simulink model "hrg_wa_v4_bitstream"  (R2025a)
settings: Solver=ode4  StartTime=0.0  StopTime=wl_stop  FixedStep=wl_Tp  RelTol=1e-3
PostLoadFcn:
  | addpath(fileparts(fileparts(get_param('hrg_wa_v4_bitstream','FileName')))); wl_setup(getVariable(get_param('hrg_wa_v4_bitstream','ModelWorkspace'),'wl_saved_configuration'));
model workspace (MAT data in the model file):
  wl_saved_configuration.stage = 4
  wl_saved_configuration.name = 'hrg_wa_v4_bitstream'
  wl_saved_configuration.head.sourceProfile = 'C:\Users\11725\Desktop\HRG_WA\HRG_WA_simulink\..\HRG_WA_Digital_ASIC_MATLAB_v4_6_5_FRP_validation_fix\HRG_WA\config\head_default.json'
  wl_saved_configuration.head.measurementStatus = 'assumed, not a measured head'
  wl_saved_configuration.head.f0 = 5000
  wl_saved_configuration.head.Q = 2000000
  wl_saved_configuration.head.bryan = 0.277
  wl_saved_configuration.head.gamma = 0.00785398163397
  wl_saved_configuration.head.dgamma = 0.00025
  wl_saved_configuration.head.dampingAxis = 0.296705972839
  wl_saved_configuration.head.splitHz = 0.008
  wl_saved_configuration.head.stiffnessAxis = 0.715584993318
  wl_saved_configuration.head.detuningHz = 0
  wl_saved_configuration.head.duffingHz = 0.015
  wl_saved_configuration.head.temperatureCoeff = -1.8e-05
  wl_saved_configuration.head.referenceTemperature = 25
  wl_saved_configuration.head.detect = [1  0.003; -0.002  1]
  wl_saved_configuration.head.detectPhase = [0; 0]
  wl_saved_configuration.head.drive = [1  0; 0  1]
  wl_saved_configuration.head.detectCubic = 0
  wl_saved_configuration.head.iqBits = 0
  wl_saved_configuration.head.iqFullScale = 2
  wl_saved_configuration.head.energyTarget = 1
  wl_saved_configuration.head.initialEnergy = 1
  wl_saved_configuration.head.initialTheta = 0.13962634016
  wl_saved_configuration.head.initialQuadRatio = 0
  wl_saved_configuration.head.energyKp = 0.8
  wl_saved_configuration.head.energyKi = 0.4
  wl_saved_configuration.head.quadKp = 2
  wl_saved_configuration.head.quadKi = 1
  wl_saved_configuration.head.pllKp = 0.8
  wl_saved_configuration.head.pllKi = 1
  wl_saved_configuration.head.energyLimit = 1
  wl_saved_configuration.head.quadLimit = 1
  wl_saved_configuration.head.pllLimitHz = 2
  wl_saved_configuration.head.antiWindup = 5
  wl_saved_configuration.head.loopEnable = 1
  wl_saved_configuration.head.Ts = 0.001
  wl_saved_configuration.head.rateTau = 0.00353677651315
  wl_saved_configuration.head.energyThreshold = 0.02
  wl_saved_configuration.head.angleThreshold = 0.01
  wl_saved_configuration.head.duration = 12
  wl_saved_configuration.head.omega = 1.3962634016
  wl_saved_configuration.head.virtualRate = 0
  wl_saved_configuration.head.temperature = 25
  wl_saved_configuration.head.fullStep = 2e-06
  wl_saved_configuration.fsAdc = 160000
  wl_saved_configuration.fsPlant = 640000
  wl_saved_configuration.duration = 0.04
  wl_saved_configuration.seed = 20261021
  wl_saved_configuration.massKg = 1e-06
  wl_saved_configuration.displacementM = 1e-07
  wl_saved_configuration.gapM = 5e-06
  wl_saved_configuration.c0F = 1e-12
  wl_saved_configuration.cfF = 1e-12
  wl_saved_configuration.rfOhm = 1000000000
  wl_saved_configuration.biasV = 10
  wl_saved_configuration.cvBandwidthHz = 30000
  wl_saved_configuration.pgaBandwidthHz = 30000
  wl_saved_configuration.pgaGain = 1
  wl_saved_configuration.cvEnVrtHz = 1e-08
  wl_saved_configuration.cvInArtHz = 1e-14
  wl_saved_configuration.temperatureK = 298.15
  wl_saved_configuration.pgaNoiseVrtHz = 1e-08
  wl_saved_configuration.afeOffsetV = [0; 0]
  wl_saved_configuration.afeLimitV = 1.8
  wl_saved_configuration.adcBits = 18
  wl_saved_configuration.adcFsV = 2
  wl_saved_configuration.adcOffsetV = [0; 0]
  wl_saved_configuration.adcGain = [1; 1]
  wl_saved_configuration.adcInlCubic = 0
  wl_saved_configuration.jitterRmsS = 2e-09
  wl_saved_configuration.channelSkewS = 0
  wl_saved_configuration.adcDelay = 1
  wl_saved_configuration.adcArchitecture = 'sigma_delta'
  wl_saved_configuration.cicStages = 3
  wl_saved_configuration.fir = [0.111111111111 0.222222222222 0.333333333333 0.222222222222 0.111111111111]
  wl_saved_configuration.dacBits = 16
  wl_saved_configuration.dacFsV = 2
  wl_saved_configuration.dacDelay = 1
  wl_saved_configuration.dacInlCubic = 0
  wl_saved_configuration.dacArchitecture = 'sigma_delta'
  wl_saved_configuration.driveNPerV = 1e-07
  wl_saved_configuration.driverBandwidthHz = 50000
  wl_saved_configuration.driverGain = [1; 1]
  wl_saved_configuration.driverSlewVPerS = 200000
  wl_saved_configuration.driverNoiseVrtHz = 2e-08
  wl_saved_configuration.driverLimitV = 1.8
  wl_saved_configuration.feedthroughF = 0
  wl_saved_configuration.pipelineCtrl = 3
  wl_saved_configuration.iqFractionBits = 22
  wl_saved_configuration.controlFractionBits = 22
  wl_saved_configuration.antiAliasHz = 18000
  wl_saved_configuration.noiseEnable = 1
  wl_saved_configuration.circuitEnable = 1
  wl_saved_configuration.kalman = 0
  wl_saved_configuration.online = 0
  wl_saved_configuration.frp = 0
  wl_saved_configuration.calibrationPermit = 0
  wl_saved_configuration.frpSequence = 0
  wl_saved_configuration.frpFreeze = 0
  wl_saved_configuration.frpTheta = [0; 0; 0; 0; 0; 0; 0; 0; 0]
  wl_saved_configuration.matrixApply = 0
  wl_saved_configuration.compensationApply = 0
  wl_saved_configuration.temperatureCompensate = 0
  wl_saved_configuration.temperatureBiasCoefficients = [0; 0; 0]
  wl_saved_configuration.zeroRateCertified = 0
  wl_saved_configuration.virtualRate = 0
  wl_saved_configuration.inputRate = 1.3962634016
  wl_saved_configuration.inputFrequencyHz = 0
  wl_saved_configuration.inputRateAmplitude = 0
  wl_saved_configuration.temperatureC = 25
  wl_saved_configuration.temperatureRampCPerS = 0
  wl_saved_configuration.observers = 0
  wl_saved_configuration.spectra = 0
  wl_saved_configuration.maxLogPoints = 80000
  wl_saved_configuration.sdmLeak = 0.9999
  wl_saved_configuration.sdmReferenceV = 2
  wl_saved_configuration.tdmEnable = 0
  wl_saved_configuration.knownPhaseCalibrationRad = -2.63258802151
  wl_saved_configuration.virtualGainCalibration = 1.10062721786
  wl_saved_configuration.learnStartS = 0.25
  wl_saved_configuration.measurementStatus = 'assumed'
  wl_saved_configuration.scope = 'Behavioral circuit interfaces, not transistor or bit-true RTL signoff'
  wl_saved_configuration.cvEquivalentNoiseVrtHz = 3.43925722091e-07
undefined symbols (not defined in the file): wl_boxcar, wl_brownVariance, wl_c, wl_capacitance, wl_control_tick, wl_cvGain, wl_cvNoiseVariance, wl_cvTau, wl_D, wl_detectGain, wl_driverNoiseVariance, wl_fir, wl_forceGain, wl_hToV, wl_input, wl_iq_quantize, wl_J, wl_jitterVariance, wl_K, wl_mix, wl_modulate, wl_p, wl_pgaNoiseVariance, wl_q0, wl_R, wl_Ta, wl_Tc, wl_Tp, wl_v0
settings Model: Creator=11725  LastModifiedBy=11725
settings DataIOCC: SaveOutput=off
settings DebuggingCC: SignalInfNanChecking=error  AlgebraicLoopMsg=error

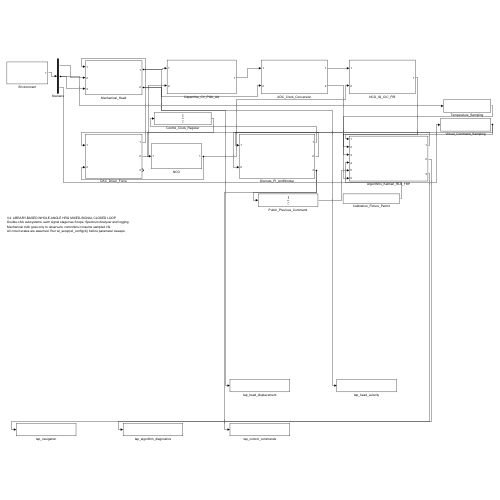
[thumbnail: Simulink's stored preview of the top-level diagram]
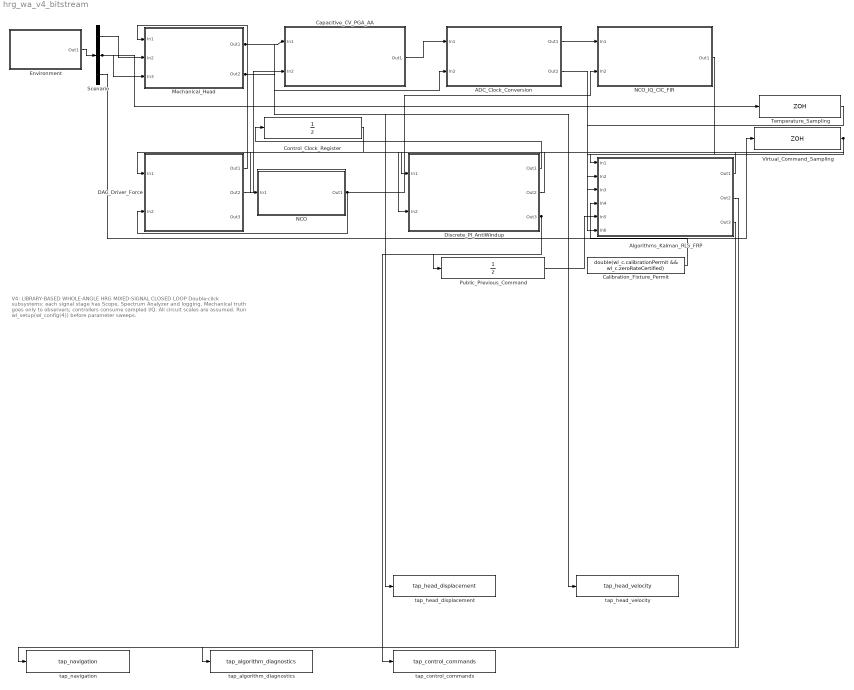
== system hrg_wa_v4_bitstream ==
  note: V4: LIBRARY-BASED WHOLE-ANGLE HRG MIXED-SIGNAL CLOSED LOOP
      | Double-click subsystems: each signal stage has Scope, Spectrum Analyzer and logging.
      | Mechanical truth goes only to observers; controllers consume sampled I/Q.
      | All circuit scales are assumed. Run wl_setup(wl_config(4)) before parameter sweeps.
  ADC_Clock_Conversion : Subsystem
  Algorithms_Kalman_RLS_FRP : Subsystem
  Calibration_Fixture_Permit : Constant  Value=double(wl_c.calibrationPermit && wl_c.zeroRateCertified)
  Capacitive_CV_PGA_AA : Subsystem
  Control_Clock_Register : UnitDelay  InitialCondition=zeros(4,1)  SampleTime=wl_Tc  HasFrameUpgradeWarning=on
  DAC_Driver_Force : Subsystem
  Discrete_PI_AntiWindup : Subsystem
  Environment : Subsystem
  Mechanical_Head : Subsystem
  NCO : Subsystem
  NCO_IQ_CIC_FIR : Subsystem
  Public_Previous_Command : UnitDelay  InitialCondition=zeros(3,1)  SampleTime=wl_Tc  HasFrameUpgradeWarning=on
  Scenario : Demux  Outputs=[2 1 1]
  Temperature_Sampling : ZeroOrderHold  SampleTime=wl_Tc
  Virtual_Command_Sampling : ZeroOrderHold  SampleTime=wl_Tc
  tap_algorithm_diagnostics : ToWorkspace  VariableName=tap_algorithm_diagnostics  SaveFormat=Timeseries  SampleTime=-1
      settings: MaxDataPoints=80000
  tap_control_commands : ToWorkspace  VariableName=tap_control_commands  SaveFormat=Timeseries  SampleTime=-1
      settings: MaxDataPoints=80000
  tap_head_displacement : ToWorkspace  VariableName=tap_head_displacement  SaveFormat=Timeseries  SampleTime=-1
      settings: MaxDataPoints=80000
  tap_head_velocity : ToWorkspace  VariableName=tap_head_velocity  SaveFormat=Timeseries  SampleTime=-1
      settings: MaxDataPoints=80000
  tap_navigation : ToWorkspace  VariableName=tap_navigation  SaveFormat=Timeseries  SampleTime=-1
      settings: MaxDataPoints=80000
  wires:
  Environment/1(Out1) -> Scenario/1
  Scenario/1 -> Mechanical_Head/2(In2)
  Scenario/2 -> Mechanical_Head/3(In3), Temperature_Sampling/1
  DAC_Driver_Force/1(Out1) -> Mechanical_Head/1(In1)
  Mechanical_Head/1(Out1) -> Capacitive_CV_PGA_AA/1(In1), tap_head_displacement/1
  DAC_Driver_Force/2(Out2) -> Capacitive_CV_PGA_AA/2(In2)
  Capacitive_CV_PGA_AA/1(Out1) -> ADC_Clock_Conversion/1(In1)
  Mechanical_Head/2(Out2) -> ADC_Clock_Conversion/2(In2), tap_head_velocity/1
  ADC_Clock_Conversion/1(Out1) -> NCO_IQ_CIC_FIR/1(In1)
  NCO/1(Out1) -> NCO_IQ_CIC_FIR/2(In2), DAC_Driver_Force/2(In2)
  NCO_IQ_CIC_FIR/1(Out1) -> Algorithms_Kalman_RLS_FRP/1(In1)
  Scenario/3 -> Virtual_Command_Sampling/1
  Temperature_Sampling/1 -> Algorithms_Kalman_RLS_FRP/2(In2)
  Virtual_Command_Sampling/1 -> Algorithms_Kalman_RLS_FRP/3(In3), Discrete_PI_AntiWindup/2(In2)
  Calibration_Fixture_Permit/1 -> Algorithms_Kalman_RLS_FRP/4(In4)
  Discrete_PI_AntiWindup/3(Out3) -> Public_Previous_Command/1, tap_control_commands/1
  Public_Previous_Command/1 -> Algorithms_Kalman_RLS_FRP/5(In5)
  Algorithms_Kalman_RLS_FRP/1(Out1) -> Discrete_PI_AntiWindup/1(In1)
  Discrete_PI_AntiWindup/2(Out2) -> NCO/1(In1)
  Discrete_PI_AntiWindup/1(Out1) -> Control_Clock_Register/1
  Control_Clock_Register/1 -> DAC_Driver_Force/1(In1)
  ADC_Clock_Conversion/2(Out2) -> Algorithms_Kalman_RLS_FRP/6(In6)
  Algorithms_Kalman_RLS_FRP/2(Out2) -> tap_navigation/1
  Algorithms_Kalman_RLS_FRP/3(Out3) -> tap_algorithm_diagnostics/1

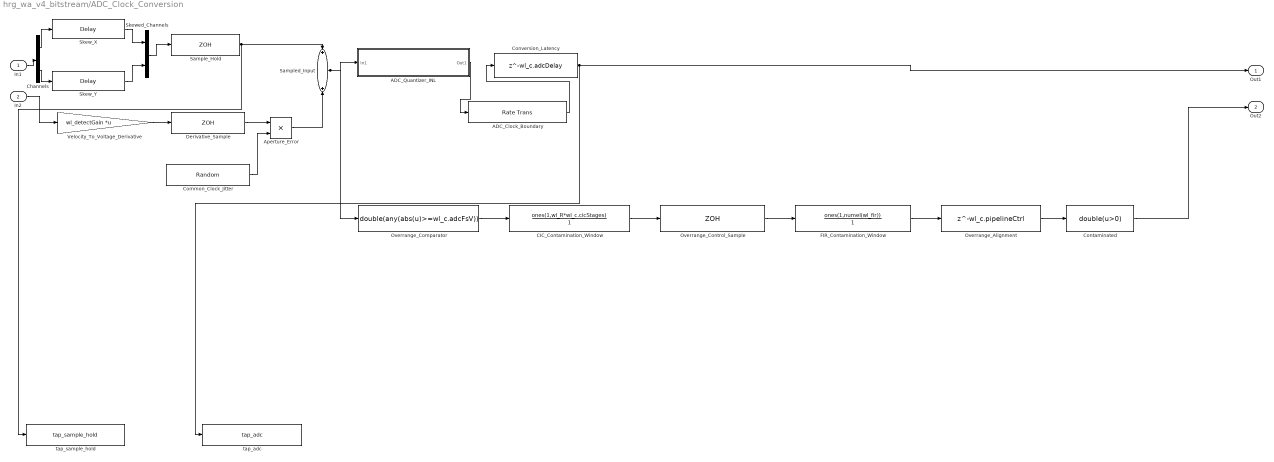
== system hrg_wa_v4_bitstream/ADC_Clock_Conversion ==
  In1 : Inport
  In2 : Inport  Port=2
  ADC_Clock_Boundary : RateTransition  Integrity=off  Deterministic=off  OutPortSampleTime=wl_Ta
  ADC_Quantizer_INL : Subsystem
  Aperture_Error : Product
  CIC_Contamination_Window : DiscreteFilter  Numerator=ones(1,wl_R*wl_c.cicStages)  Denominator=1  SampleTime=wl_Ta
  Channels : Demux  Outputs=2
  Common_Clock_Jitter : RandomNumber  Variance=wl_jitterVariance  Seed=wl_c.seed+621  SampleTime=wl_Ta
  Contaminated : MATLABFcn  MATLABFcn=double(u>0)  OutputDimensions=1
  Conversion_Latency : Delay  DelayLength=wl_c.adcDelay  InitialCondition=0  SampleTime=wl_Ta
  Derivative_Sample : ZeroOrderHold  SampleTime=wl_Ta
  FIR_Contamination_Window : DiscreteFilter  Numerator=ones(1,numel(wl_fir))  Denominator=1  SampleTime=wl_Tc
  Overrange_Alignment : Delay  DelayLength=wl_c.pipelineCtrl  InitialCondition=0  SampleTime=wl_Tc
  Overrange_Comparator : MATLABFcn  MATLABFcn=double(any(abs(u)>=wl_c.adcFsV))  OutputDimensions=1
  Overrange_Control_Sample : ZeroOrderHold  SampleTime=wl_Tc
  Sample_Hold : ZeroOrderHold  SampleTime=wl_Ta
  Sampled_Input : Sum
  Skew_X : TransportDelay  DelayTime=max(-wl_c.channelSkewS,0)
  Skew_Y : TransportDelay  DelayTime=max(wl_c.channelSkewS,0)
  Skewed_Channels : Mux  Inputs=2
  Velocity_To_Voltage_Derivative : Gain  Gain=wl_detectGain  Multiplication=Matrix(K*u)
  tap_adc : ToWorkspace  VariableName=tap_adc  SaveFormat=Timeseries  SampleTime=-1
      settings: MaxDataPoints=80000
  tap_sample_hold : ToWorkspace  VariableName=tap_sample_hold  SaveFormat=Timeseries  SampleTime=-1
      settings: MaxDataPoints=80000
  Out1 : Outport
  Out2 : Outport  Port=2
  wires:
  In1/1 -> Channels/1
  Channels/1 -> Skew_X/1
  Channels/2 -> Skew_Y/1
  Skew_X/1 -> Skewed_Channels/1
  Skew_Y/1 -> Skewed_Channels/2
  Skewed_Channels/1 -> Sample_Hold/1
  In2/1 -> Velocity_To_Voltage_Derivative/1
  Velocity_To_Voltage_Derivative/1 -> Derivative_Sample/1
  Derivative_Sample/1 -> Aperture_Error/1
  Common_Clock_Jitter/1 -> Aperture_Error/2
  Sample_Hold/1 -> Sampled_Input/1, tap_sample_hold/1
  Aperture_Error/1 -> Sampled_Input/2
  Sampled_Input/1 -> ADC_Quantizer_INL/1(In1), Overrange_Comparator/1
  ADC_Quantizer_INL/1(Out1) -> ADC_Clock_Boundary/1
  ADC_Clock_Boundary/1 -> Conversion_Latency/1
  Conversion_Latency/1 -> Out1/1, tap_adc/1
  Overrange_Comparator/1 -> CIC_Contamination_Window/1
  CIC_Contamination_Window/1 -> Overrange_Control_Sample/1
  Overrange_Control_Sample/1 -> FIR_Contamination_Window/1
  FIR_Contamination_Window/1 -> Overrange_Alignment/1
  Overrange_Alignment/1 -> Contaminated/1
  Contaminated/1 -> Out2/1

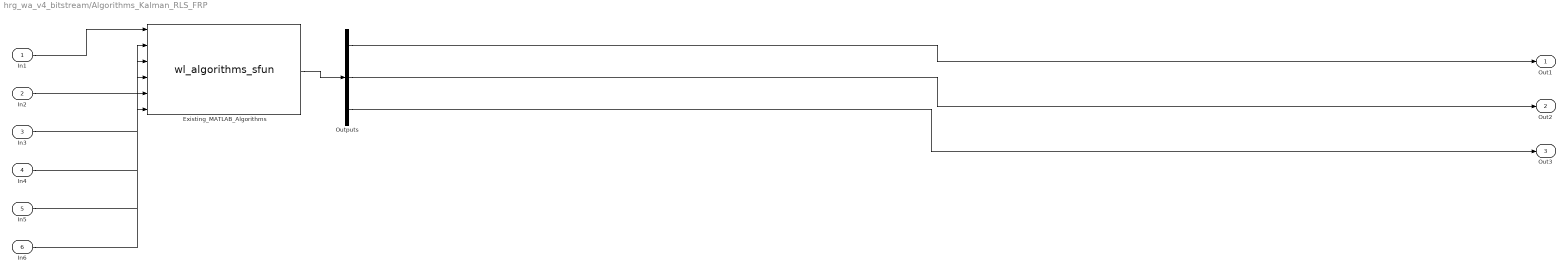
== system hrg_wa_v4_bitstream/Algorithms_Kalman_RLS_FRP ==
  In1 : Inport
  In2 : Inport  Port=2
  In3 : Inport  Port=3
  In4 : Inport  Port=4
  In5 : Inport  Port=5
  In6 : Inport  Port=6
  Existing_MATLAB_Algorithms : M-S-Function  FunctionName=wl_algorithms_sfun  Parameters=wl_c
  Outputs : Demux  Outputs=[10 4 21]
  Out1 : Outport
  Out2 : Outport  Port=2
  Out3 : Outport  Port=3
  wires:
  In1/1 -> Existing_MATLAB_Algorithms/1
  In2/1 -> Existing_MATLAB_Algorithms/2
  In3/1 -> Existing_MATLAB_Algorithms/3
  In4/1 -> Existing_MATLAB_Algorithms/4
  In5/1 -> Existing_MATLAB_Algorithms/5
  In6/1 -> Existing_MATLAB_Algorithms/6
  Existing_MATLAB_Algorithms/1 -> Outputs/1
  Outputs/1 -> Out1/1
  Outputs/2 -> Out2/1
  Outputs/3 -> Out3/1

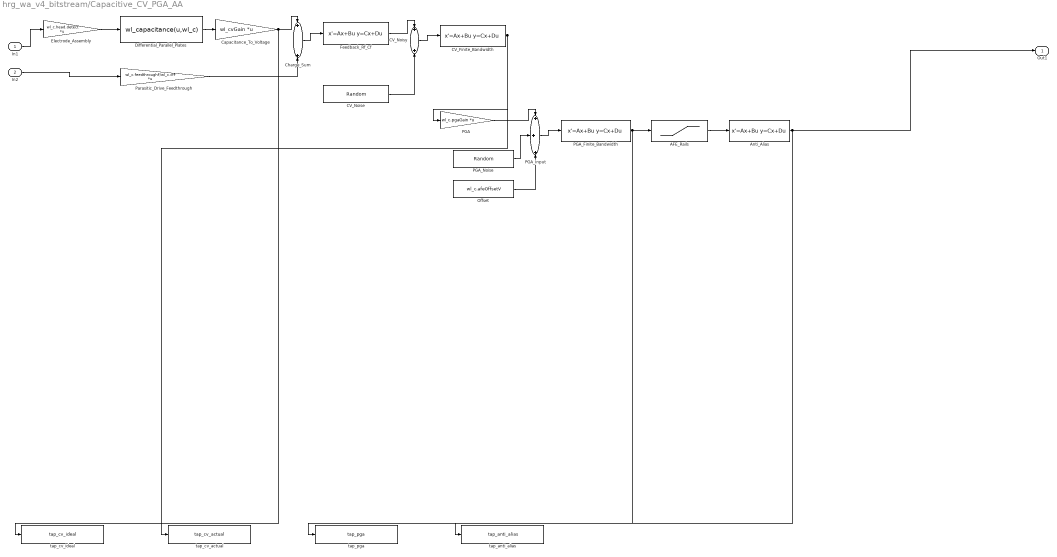
== system hrg_wa_v4_bitstream/Capacitive_CV_PGA_AA ==
  In1 : Inport
  In2 : Inport  Port=2
  AFE_Rails : Saturate  UpperLimit=wl_c.afeLimitV  LowerLimit=-wl_c.afeLimitV
  Anti_Alias : StateSpace  A=-2*pi*wl_c.antiAliasHz*eye(2)  B=2*pi*wl_c.antiAliasHz*eye(2)  C=eye(2)  D=zeros(2)  InitialCondition=0
  CV_Finite_Bandwidth : StateSpace  A=-2*pi*wl_c.cvBandwidthHz*eye(2)  B=2*pi*wl_c.cvBandwidthHz*eye(2)  C=eye(2)  D=zeros(2)  InitialCondition=0
  CV_Noise : RandomNumber  Mean=[0;0]  Variance=wl_cvNoiseVariance*[1;1]  Seed=[wl_c.seed+601;wl_c.seed+602]  SampleTime=wl_Tp
  CV_Noisy : Sum
  Capacitance_To_Voltage : Gain  Gain=wl_cvGain  Multiplication=Matrix(K*u)
  Charge_Sum : Sum
  Differential_Parallel_Plates : MATLABFcn  MATLABFcn=wl_capacitance(u,wl_c)  OutputDimensions=2
  Electrode_Assembly : Gain  Gain=wl_c.head.detect  Multiplication=Matrix(K*u)
  Feedback_Rf_Cf : StateSpace  A=-eye(2)/wl_cvTau  B=eye(2)/wl_cvTau  C=-eye(2)  D=eye(2)  InitialCondition=0
  Offset : Constant  Value=wl_c.afeOffsetV
  PGA : Gain  Gain=wl_c.pgaGain  Multiplication=Matrix(K*u)
  PGA_Finite_Bandwidth : StateSpace  A=-2*pi*wl_c.pgaBandwidthHz*eye(2)  B=2*pi*wl_c.pgaBandwidthHz*eye(2)  C=eye(2)  D=zeros(2)  InitialCondition=0
  PGA_Input : Sum  Inputs=+++
  PGA_Noise : RandomNumber  Mean=[0;0]  Variance=wl_pgaNoiseVariance*[1;1]  Seed=[wl_c.seed+611;wl_c.seed+612]  SampleTime=wl_Tp
  Parasitic_Drive_Feedthrough : Gain  Gain=wl_c.feedthroughF/wl_c.cfF  Multiplication=Matrix(K*u)
  tap_anti_alias : ToWorkspace  VariableName=tap_anti_alias  SaveFormat=Timeseries  SampleTime=-1
      settings: MaxDataPoints=80000
  tap_cv_actual : ToWorkspace  VariableName=tap_cv_actual  SaveFormat=Timeseries  SampleTime=-1
      settings: MaxDataPoints=80000
  tap_cv_ideal : ToWorkspace  VariableName=tap_cv_ideal  SaveFormat=Timeseries  SampleTime=-1
      settings: MaxDataPoints=80000
  tap_pga : ToWorkspace  VariableName=tap_pga  SaveFormat=Timeseries  SampleTime=-1
      settings: MaxDataPoints=80000
  Out1 : Outport
  wires:
  In1/1 -> Electrode_Assembly/1
  Electrode_Assembly/1 -> Differential_Parallel_Plates/1
  Differential_Parallel_Plates/1 -> Capacitance_To_Voltage/1
  In2/1 -> Parasitic_Drive_Feedthrough/1
  Capacitance_To_Voltage/1 -> Charge_Sum/1, tap_cv_ideal/1
  Parasitic_Drive_Feedthrough/1 -> Charge_Sum/2
  Charge_Sum/1 -> Feedback_Rf_Cf/1
  Feedback_Rf_Cf/1 -> CV_Noisy/1
  CV_Noise/1 -> CV_Noisy/2
  CV_Noisy/1 -> CV_Finite_Bandwidth/1
  CV_Finite_Bandwidth/1 -> PGA/1, tap_cv_actual/1
  PGA/1 -> PGA_Input/1
  PGA_Noise/1 -> PGA_Input/2
  Offset/1 -> PGA_Input/3
  PGA_Input/1 -> PGA_Finite_Bandwidth/1
  PGA_Finite_Bandwidth/1 -> AFE_Rails/1, tap_pga/1
  AFE_Rails/1 -> Anti_Alias/1
  Anti_Alias/1 -> Out1/1, tap_anti_alias/1

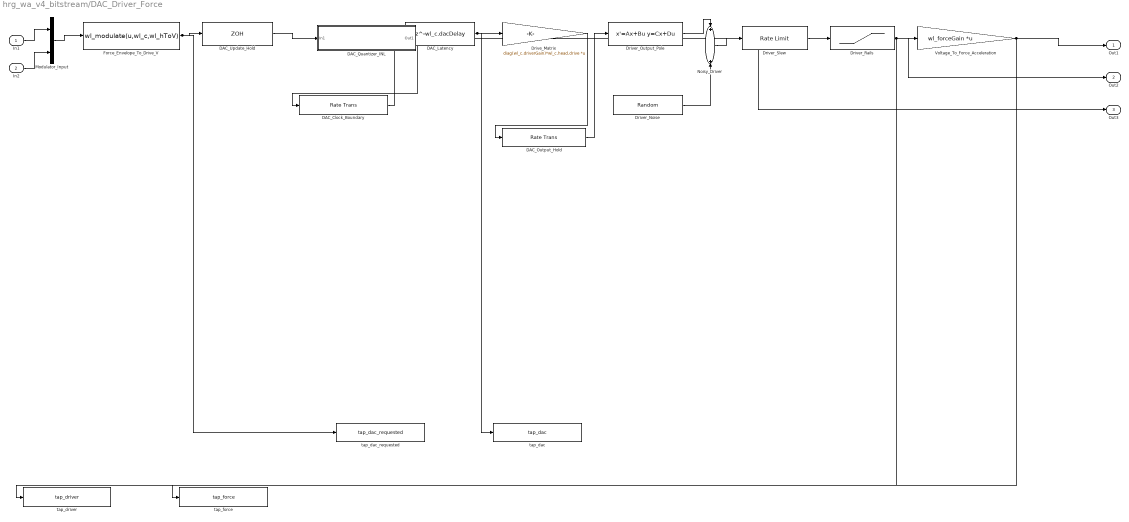
== system hrg_wa_v4_bitstream/DAC_Driver_Force ==
  In1 : Inport
  In2 : Inport  Port=2
  DAC_Clock_Boundary : RateTransition  Integrity=off  Deterministic=off  OutPortSampleTime=wl_Ta
  DAC_Latency : Delay  DelayLength=wl_c.dacDelay  InitialCondition=0  SampleTime=wl_Ta
  DAC_Output_Hold : RateTransition  Integrity=off  Deterministic=off  OutPortSampleTime=0
  DAC_Quantizer_INL : Subsystem
  DAC_Update_Hold : ZeroOrderHold  SampleTime=wl_Ta
  Drive_Matrix : Gain  Gain=diag(wl_c.driverGain)*wl_c.head.drive  Multiplication=Matrix(K*u)
  Driver_Noise : RandomNumber  Mean=[0;0]  Variance=wl_driverNoiseVariance*[1;1]  Seed=[wl_c.seed+631;wl_c.seed+632]  SampleTime=wl_Tp
  Driver_Output_Pole : StateSpace  A=-2*pi*wl_c.driverBandwidthHz*eye(2)  B=2*pi*wl_c.driverBandwidthHz*eye(2)  C=eye(2)  D=zeros(2)  InitialCondition=0
  Driver_Rails : Saturate  UpperLimit=wl_c.driverLimitV  LowerLimit=-wl_c.driverLimitV
  Driver_Slew : RateLimiter  RisingSlewLimit=wl_c.driverSlewVPerS  FallingSlewLimit=-wl_c.driverSlewVPerS  SampleTimeMode=inherited
  Force_Envelope_To_Drive_V : MATLABFcn  MATLABFcn=wl_modulate(u,wl_c,wl_hToV)  OutputDimensions=2
  Modulator_Input : Mux  Inputs=2
  Noisy_Driver : Sum
  Voltage_To_Force_Acceleration : Gain  Gain=wl_forceGain  Multiplication=Matrix(K*u)
  tap_dac : ToWorkspace  VariableName=tap_dac  SaveFormat=Timeseries  SampleTime=-1
      settings: MaxDataPoints=80000
  tap_dac_requested : ToWorkspace  VariableName=tap_dac_requested  SaveFormat=Timeseries  SampleTime=-1
      settings: MaxDataPoints=80000
  tap_driver : ToWorkspace  VariableName=tap_driver  SaveFormat=Timeseries  SampleTime=-1
      settings: MaxDataPoints=80000
  tap_force : ToWorkspace  VariableName=tap_force  SaveFormat=Timeseries  SampleTime=-1
      settings: MaxDataPoints=80000
  Out1 : Outport
  Out2 : Outport  Port=2
  Out3 : Outport  Port=3
  wires:
  In1/1 -> Modulator_Input/1
  In2/1 -> Modulator_Input/2
  Modulator_Input/1 -> Force_Envelope_To_Drive_V/1
  Force_Envelope_To_Drive_V/1 -> DAC_Update_Hold/1, tap_dac_requested/1
  DAC_Update_Hold/1 -> DAC_Quantizer_INL/1(In1)
  DAC_Quantizer_INL/1(Out1) -> DAC_Clock_Boundary/1, Out3/1
  DAC_Clock_Boundary/1 -> DAC_Latency/1
  DAC_Latency/1 -> Drive_Matrix/1, tap_dac/1
  Drive_Matrix/1 -> DAC_Output_Hold/1
  DAC_Output_Hold/1 -> Driver_Output_Pole/1
  Driver_Output_Pole/1 -> Noisy_Driver/1
  Driver_Noise/1 -> Noisy_Driver/2
  Noisy_Driver/1 -> Driver_Slew/1
  Driver_Slew/1 -> Driver_Rails/1
  Driver_Rails/1 -> Voltage_To_Force_Acceleration/1, Out2/1, tap_driver/1
  Voltage_To_Force_Acceleration/1 -> Out1/1, tap_force/1

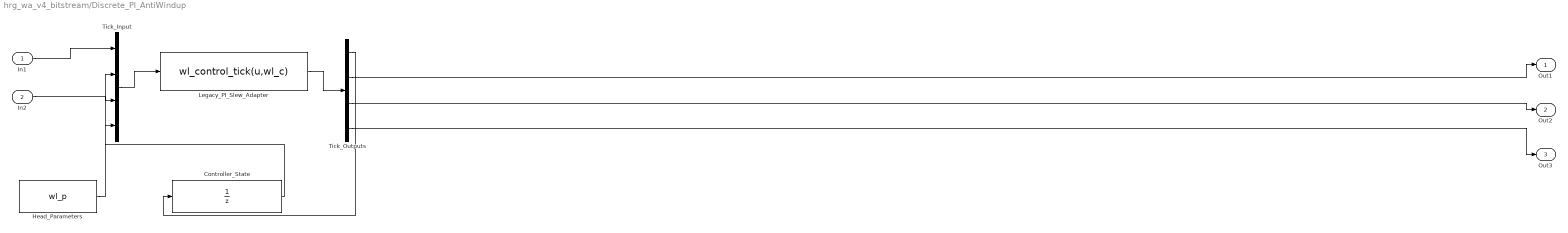
== system hrg_wa_v4_bitstream/Discrete_PI_AntiWindup ==
  In1 : Inport
  In2 : Inport  Port=2
  Controller_State : UnitDelay  InitialCondition=zeros(6,1)  SampleTime=wl_Tc  HasFrameUpgradeWarning=on
  Head_Parameters : Constant  Value=wl_p
  Legacy_PI_Slew_Adapter : MATLABFcn  MATLABFcn=wl_control_tick(u,wl_c)  OutputDimensions=14
  Tick_Input : Mux
  Tick_Outputs : Demux  Outputs=[6 4 1 3]
  Out1 : Outport
  Out2 : Outport  Port=2
  Out3 : Outport  Port=3
  wires:
  In1/1 -> Tick_Input/1
  Controller_State/1 -> Tick_Input/2
  In2/1 -> Tick_Input/3
  Head_Parameters/1 -> Tick_Input/4
  Tick_Input/1 -> Legacy_PI_Slew_Adapter/1
  Legacy_PI_Slew_Adapter/1 -> Tick_Outputs/1
  Tick_Outputs/1 -> Controller_State/1
  Tick_Outputs/2 -> Out1/1
  Tick_Outputs/3 -> Out2/1
  Tick_Outputs/4 -> Out3/1

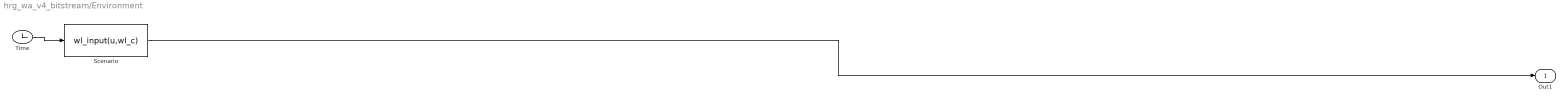
== system hrg_wa_v4_bitstream/Environment ==
  Scenario : MATLABFcn  MATLABFcn=wl_input(u,wl_c)  OutputDimensions=4
  Time : Clock
  Out1 : Outport
  wires:
  Time/1 -> Scenario/1
  Scenario/1 -> Out1/1

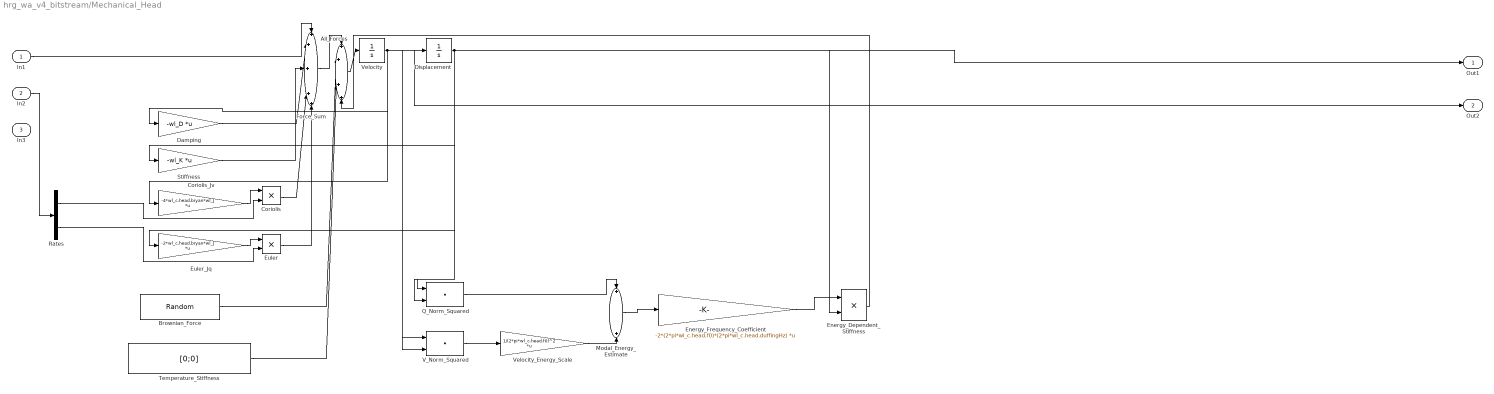
== system hrg_wa_v4_bitstream/Mechanical_Head ==
  In1 : Inport
  In2 : Inport  Port=2
  In3 : Inport  Port=3
  All_Forces : Sum  Inputs=++++
  Brownian_Force : RandomNumber  Mean=[0;0]  Variance=wl_brownVariance*[1;1]  Seed=[wl_c.seed+501;wl_c.seed+502]  SampleTime=wl_Tp
  Coriolis : Product
  Coriolis_Jv : Gain  Gain=-4*wl_c.head.bryan*wl_J  Multiplication=Matrix(K*u)
  Damping : Gain  Gain=-wl_D  Multiplication=Matrix(K*u)
  Displacement : Integrator  InitialCondition=wl_q0
  Energy_Dependent_Stiffness : Product
  Energy_Frequency_Coefficient : Gain  Gain=-2*(2*pi*wl_c.head.f0)*(2*pi*wl_c.head.duffingHz)  Multiplication=Matrix(K*u)
  Euler : Product
  Euler_Jq : Gain  Gain=-2*wl_c.head.bryan*wl_J  Multiplication=Matrix(K*u)
  Force_Sum : Sum  Inputs=+++++
  Modal_Energy_Estimate : Sum
  Q_Norm_Squared : DotProduct  OutDataTypeStr=Inherit: Inherit via internal rule
  Rates : Demux  Outputs=2
  Stiffness : Gain  Gain=-wl_K  Multiplication=Matrix(K*u)
  Temperature_Stiffness : Constant  Value=[0;0]
  V_Norm_Squared : DotProduct  OutDataTypeStr=Inherit: Inherit via internal rule
  Velocity : Integrator  InitialCondition=wl_v0
  Velocity_Energy_Scale : Gain  Gain=1/(2*pi*wl_c.head.f0)^2  Multiplication=Matrix(K*u)
  Out1 : Outport
  Out2 : Outport  Port=2
  wires:
  In1/1 -> Force_Sum/1
  Velocity/1 -> Damping/1, Coriolis_Jv/1, V_Norm_Squared/1, V_Norm_Squared/2, Displacement/1, Out2/1
  Damping/1 -> Force_Sum/2
  Displacement/1 -> Stiffness/1, Euler_Jq/1, Q_Norm_Squared/1, Q_Norm_Squared/2, Energy_Dependent_Stiffness/2, Out1/1
  Stiffness/1 -> Force_Sum/3
  In2/1 -> Rates/1
  Coriolis_Jv/1 -> Coriolis/1
  Rates/1 -> Coriolis/2
  Euler_Jq/1 -> Euler/1
  Rates/2 -> Euler/2
  Coriolis/1 -> Force_Sum/4
  Euler/1 -> Force_Sum/5
  V_Norm_Squared/1 -> Velocity_Energy_Scale/1
  Q_Norm_Squared/1 -> Modal_Energy_Estimate/1
  Velocity_Energy_Scale/1 -> Modal_Energy_Estimate/2
  Modal_Energy_Estimate/1 -> Energy_Frequency_Coefficient/1
  Energy_Frequency_Coefficient/1 -> Energy_Dependent_Stiffness/1
  Energy_Dependent_Stiffness/1 -> All_Forces/4
  Force_Sum/1 -> All_Forces/1
  Brownian_Force/1 -> All_Forces/2
  Temperature_Stiffness/1 -> All_Forces/3
  All_Forces/1 -> Velocity/1

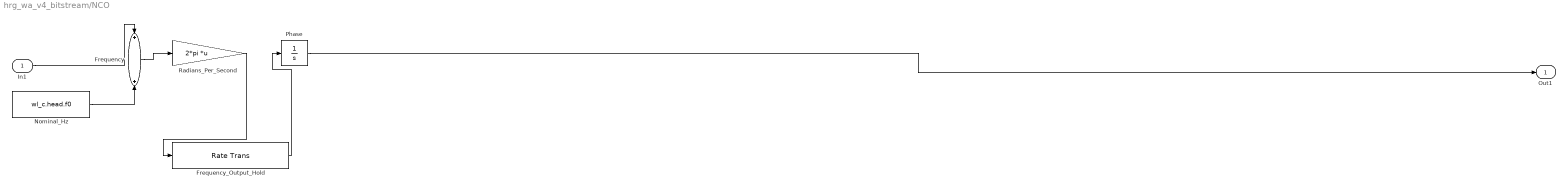
== system hrg_wa_v4_bitstream/NCO ==
  In1 : Inport
  Frequency : Sum
  Frequency_Output_Hold : RateTransition  Integrity=off  Deterministic=off  OutPortSampleTime=0
  Nominal_Hz : Constant  Value=wl_c.head.f0
  Phase : Integrator
  Radians_Per_Second : Gain  Gain=2*pi  Multiplication=Matrix(K*u)
  Out1 : Outport
  wires:
  In1/1 -> Frequency/1
  Nominal_Hz/1 -> Frequency/2
  Frequency/1 -> Radians_Per_Second/1
  Radians_Per_Second/1 -> Frequency_Output_Hold/1
  Frequency_Output_Hold/1 -> Phase/1
  Phase/1 -> Out1/1

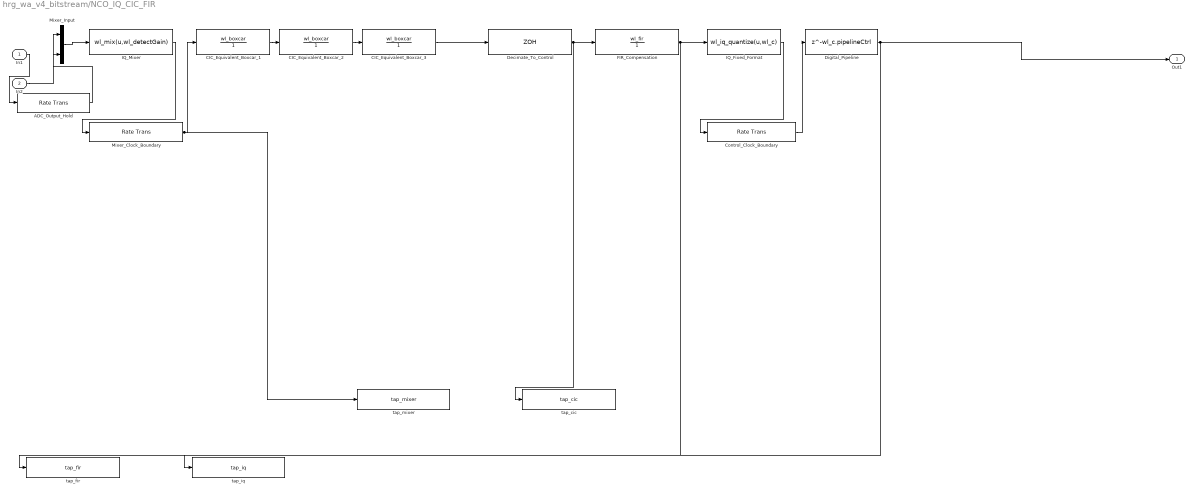
== system hrg_wa_v4_bitstream/NCO_IQ_CIC_FIR ==
  In1 : Inport
  In2 : Inport  Port=2
  ADC_Output_Hold : RateTransition  Integrity=off  Deterministic=off  OutPortSampleTime=0
  CIC_Equivalent_Boxcar_1 : DiscreteFilter  Numerator=wl_boxcar  Denominator=1  SampleTime=wl_Ta
  CIC_Equivalent_Boxcar_2 : DiscreteFilter  Numerator=wl_boxcar  Denominator=1  SampleTime=wl_Ta
  CIC_Equivalent_Boxcar_3 : DiscreteFilter  Numerator=wl_boxcar  Denominator=1  SampleTime=wl_Ta
  Control_Clock_Boundary : RateTransition  Integrity=off  Deterministic=off  OutPortSampleTime=wl_Tc
  Decimate_To_Control : ZeroOrderHold  SampleTime=wl_Tc
  Digital_Pipeline : Delay  DelayLength=wl_c.pipelineCtrl  InitialCondition=0  SampleTime=wl_Tc
  FIR_Compensation : DiscreteFilter  Numerator=wl_fir  Denominator=1  SampleTime=wl_Tc
  IQ_Fixed_Format : MATLABFcn  MATLABFcn=wl_iq_quantize(u,wl_c)  OutputDimensions=4
  IQ_Mixer : MATLABFcn  MATLABFcn=wl_mix(u,wl_detectGain)  OutputDimensions=4
  Mixer_Clock_Boundary : RateTransition  Integrity=off  Deterministic=off  OutPortSampleTime=wl_Ta
  Mixer_Input : Mux  Inputs=2
  tap_cic : ToWorkspace  VariableName=tap_cic  SaveFormat=Timeseries  SampleTime=-1
      settings: MaxDataPoints=80000
  tap_fir : ToWorkspace  VariableName=tap_fir  SaveFormat=Timeseries  SampleTime=-1
      settings: MaxDataPoints=80000
  tap_iq : ToWorkspace  VariableName=tap_iq  SaveFormat=Timeseries  SampleTime=-1
      settings: MaxDataPoints=80000
  tap_mixer : ToWorkspace  VariableName=tap_mixer  SaveFormat=Timeseries  SampleTime=-1
      settings: MaxDataPoints=80000
  Out1 : Outport
  wires:
  In1/1 -> ADC_Output_Hold/1
  ADC_Output_Hold/1 -> Mixer_Input/1
  In2/1 -> Mixer_Input/2
  Mixer_Input/1 -> IQ_Mixer/1
  IQ_Mixer/1 -> Mixer_Clock_Boundary/1
  Mixer_Clock_Boundary/1 -> CIC_Equivalent_Boxcar_1/1, tap_mixer/1
  CIC_Equivalent_Boxcar_1/1 -> CIC_Equivalent_Boxcar_2/1
  CIC_Equivalent_Boxcar_2/1 -> CIC_Equivalent_Boxcar_3/1
  CIC_Equivalent_Boxcar_3/1 -> Decimate_To_Control/1
  Decimate_To_Control/1 -> FIR_Compensation/1, tap_cic/1
  FIR_Compensation/1 -> IQ_Fixed_Format/1, tap_fir/1
  IQ_Fixed_Format/1 -> Control_Clock_Boundary/1
  Control_Clock_Boundary/1 -> Digital_Pipeline/1
  Digital_Pipeline/1 -> Out1/1, tap_iq/1

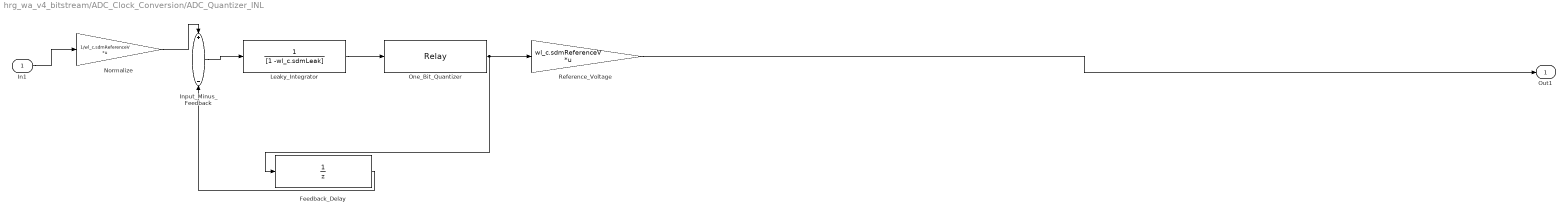
== system hrg_wa_v4_bitstream/ADC_Clock_Conversion/ADC_Quantizer_INL ==
  In1 : Inport
  Feedback_Delay : UnitDelay  SampleTime=wl_Ta  HasFrameUpgradeWarning=on
  Input_Minus_Feedback : Sum  Inputs=+-
  Leaky_Integrator : DiscreteFilter  Numerator=1  Denominator=[1 -wl_c.sdmLeak]  SampleTime=wl_Ta
  Normalize : Gain  Gain=1/wl_c.sdmReferenceV  Multiplication=Matrix(K*u)
  One_Bit_Quantizer : Relay  OnSwitchValue=0  OffSwitchValue=0  OffOutputValue=-1
  Reference_Voltage : Gain  Gain=wl_c.sdmReferenceV  Multiplication=Matrix(K*u)
  Out1 : Outport
  wires:
  In1/1 -> Normalize/1
  Normalize/1 -> Input_Minus_Feedback/1
  Input_Minus_Feedback/1 -> Leaky_Integrator/1
  Leaky_Integrator/1 -> One_Bit_Quantizer/1
  One_Bit_Quantizer/1 -> Feedback_Delay/1, Reference_Voltage/1
  Feedback_Delay/1 -> Input_Minus_Feedback/2
  Reference_Voltage/1 -> Out1/1

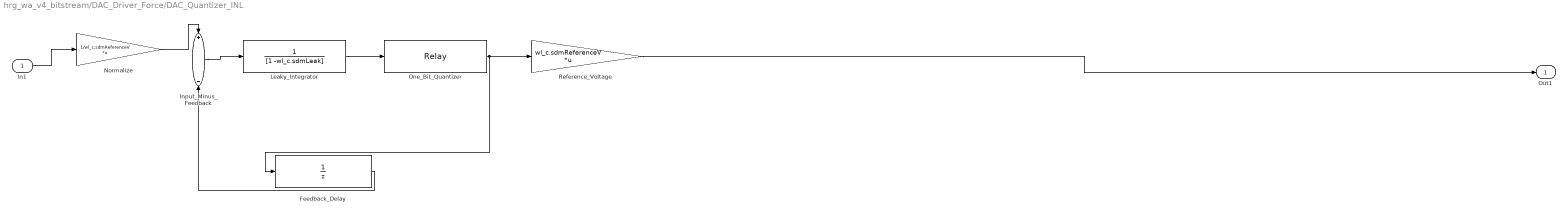
== system hrg_wa_v4_bitstream/DAC_Driver_Force/DAC_Quantizer_INL ==
  In1 : Inport
  Feedback_Delay : UnitDelay  SampleTime=wl_Ta  HasFrameUpgradeWarning=on
  Input_Minus_Feedback : Sum  Inputs=+-
  Leaky_Integrator : DiscreteFilter  Numerator=1  Denominator=[1 -wl_c.sdmLeak]  SampleTime=wl_Ta
  Normalize : Gain  Gain=1/wl_c.sdmReferenceV  Multiplication=Matrix(K*u)
  One_Bit_Quantizer : Relay  OnSwitchValue=0  OffSwitchValue=0  OffOutputValue=-1
  Reference_Voltage : Gain  Gain=wl_c.sdmReferenceV  Multiplication=Matrix(K*u)
  Out1 : Outport
  wires:
  In1/1 -> Normalize/1
  Normalize/1 -> Input_Minus_Feedback/1
  Input_Minus_Feedback/1 -> Leaky_Integrator/1
  Leaky_Integrator/1 -> One_Bit_Quantizer/1
  One_Bit_Quantizer/1 -> Feedback_Delay/1, Reference_Voltage/1
  Feedback_Delay/1 -> Input_Minus_Feedback/2
  Reference_Voltage/1 -> Out1/1
